simulink model "SpaceRobot"  (R2025b)
settings: Solver=ode4  StartTime=0.0  StopTime=8.5  FixedStep=0.01  RelTol=1e-5  AbsTol=1e-6
undefined symbols (not defined in the file or in its folder): d_safe, isdone_init, reward_init, Ts_agent, X, Y, Z
libraries: sm_lib x53, nesl_utility x34, rllib x1, sharedutil x1
(part 1 of 2)
settings Model: Creator=Deermste  LastModifiedBy=Deermste
settings ExplorerConfigSet: InternalSimMechanicsExplorerSettings="<ExplorerConfiguration><canonicalview>default</canonicalview><TilePanel><TileInfo><Tiles Columns=\"1\" Count=\"1\" Height=\"297\" Rows=\"1\" Width=\"493\"><Row Weight=\"1\"/><Column Weight=\"1\"/><Tile Height=\"1\" Width=\"1\" X=\"0\" Y=\"0\"/></Tiles></TileInfo><SceneInfo><SceneViewer><IsThisViewStd><IsStandardView>off</IsStandardView><StandardViewName>Front</StandardViewName></IsThisViewStd><BGColor><R>1</R><G>1</G><B>1</B><A>1</A></BGColor><Camera><DoPerspective>off</DoPerspective><Position><X>1.8433594980602974</X><Y>0.042277202971402056</Y><Z>13.278475546002786</Z></Position><Center><X>1.8433594980602974</X><Y>0.042277202971402056</Y><Z>0</Z></Center><Up><X>0</X><Y>1</Y><Z>0</Z></Up><XLim>1.9650781003092099</XLim><YLim>1.9650781003092099</YLim><ViewLimDist>0.01</ViewLimDist></Camera></SceneViewer></SceneInfo></TilePanel><MechEditorPanel><GfxPanelCameraMap/><Cameras/><VideoCreator><IncludeTiles>All</IncludeTiles><IncludeTime>on</IncludeTime><IncludeWorldFrame>off</IncludeWorldFrame><PlaybackSpeedRatio>1</PlaybackSpeedRatio><FrameRate>30</FrameRate><FrameSize>auto</FrameSize><VideoFormat>UncompressedAVI</VideoFormat></VideoCreator></MechEditorPanel><PlaybackSettings><PlaybackSpeedFactor>1</PlaybackSpeedFactor></PlaybackSettings></ExplorerConfiguration>"
settings ConfigComp: DVMaxProcessTime=300.0  DVMaxTestCaseSteps=10000.0  DVTestSuiteOptimization=Auto  DVAbsoluteTolerance=1.0e-5  DVDefectChecker=on  DVDetectOutOfBounds=on  DVMaxViolationSteps=20.0  DVModelReferenceHarness=on  DVHarnessSource=Signal Editor  DVActiveTab=0.0

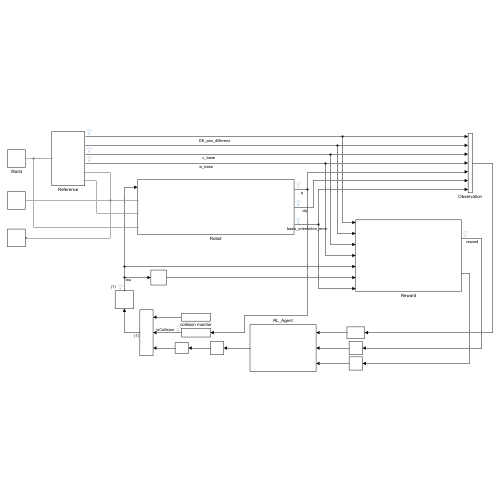
[thumbnail: Simulink's stored preview of the top-level diagram]
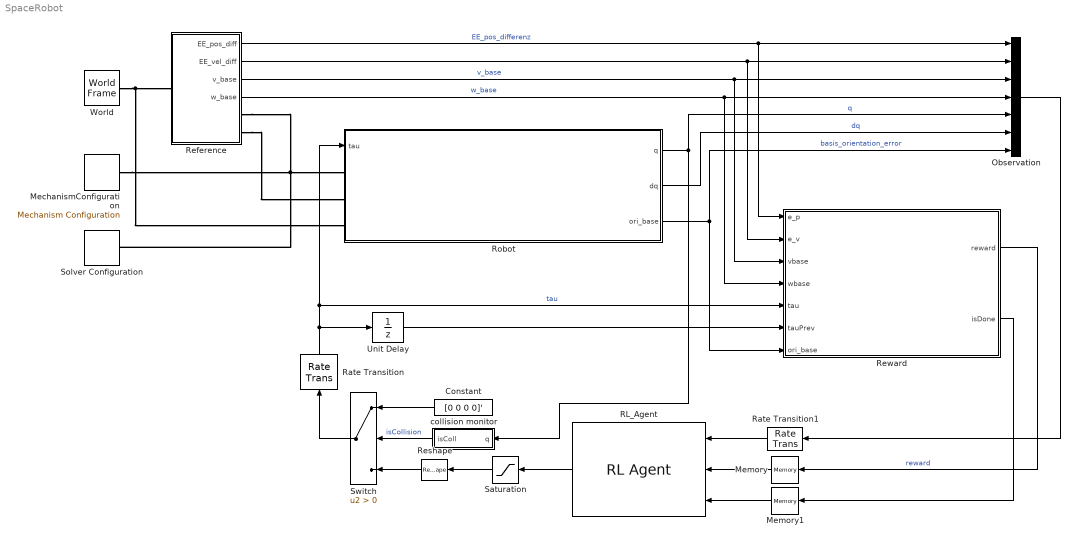
== system SpaceRobot ==
  Constant : Constant  Value=[0 0 0 0]'
  MechanismConfiguration : sm_lib/Utilities/Mechanism Configuration  UniformGravity=Constant  GravityVector=[0 0 0]  GravityVectorUnits=m/s^2  LinearizationDelta=0.001  JointModeTransitionNonlinearIterations=2
  Memory : Memory  InitialCondition=reward_init  InheritSampleTime=on
  Memory1 : Memory  InitialCondition=isdone_init  InheritSampleTime=on
  Observation : Mux  Inputs=7
  RL_Agent : rllib/RL Agent  Agent=agent  ExternalActionAsInput=off  ProvideLastAction=off  ProvideCumRwd=off  TreatAsDirectFeedthrough=on  UseStrictObservationDataTypes=off
  Rate Transition : RateTransition  OutPortSampleTime=Ts
  Rate Transition1 : RateTransition  OutPortSampleTime=Ts_agent
  Reference : Subsystem
  Reshape : Reshape  OutputDimensionality=Customize  OutputDimensions=[4, 1]
  Reward : Subsystem
  Robot : Subsystem
  Saturation : Saturate  UpperLimit=2  LowerLimit=-2
  Solver Configuration : nesl_utility/Solver Configuration  PhysicalDomain=network_engine_domain  SubClassName=solver  LeftPortType=input  RightPortType=generic  Tones=[]  Harmonics=[]  SimulateNoise=off  Profile=off  UseLocalSampling=off  EnableSwitchedLinearOptims=on  FrequencyDomain=off  UseCCode=off  RelTol=0.001  AbsTol=0.001  MinStep=1e-09  ToWorkspace=off  RevertToSquareIcSolve=off  NumHomotopyIterations=100  PhasorMode=off  PhasorModeNumHarmonics=1  ConsistencySolver=NEWTON_XTOL_AFTER_FTOL  IndexReductionMethod=DerivativeReplacement  DoDC=off  ResidualTolerance=1e-09  ConsistencyTolSource=GLOBAL  ConsistencyAbsTol=0.001  ConsistencyRelTol=0.001  ConsistencyTolFactor=0.001  UseLocalSolver=off  LocalSolverChoice=NE_BACKWARD_EULER_ADVANCER  ResolveIndetEquations=on  FunctionEvalNumThread=1  LocalSolverSampleTime=0.001  DoFixedCost=off  MaxNonlinIter=3  MaxModeIter=2  ComputeImpulses=off  ImpulseIterations=2  LinearAlgebra=auto  LinearAlgebraNumThread=0  EquationFormulation=NE_TIME_EF  DelaysMemoryBudget=1024  AutomaticFiltering=on  FilteringTimeConstant=0.001  PartitionStorageMethod=AS_NEEDED  PartitionMemoryBudget=1024  PartitionMethod=ROBUST  MultibodyUseLocalSolver=off  MultibodyLocalSolverChoice=ODE1  MultibodyLocalSolverSampleTime=0.001
  Switch : Switch  Criteria=u2 > Threshold  SaturateOnIntegerOverflow=off  InputSameDT=off
  Unit Delay : UnitDelay  InitialCondition=zeros(4,1)  SampleTime=-1  HasFrameUpgradeWarning=on
  World : sm_lib/Frames and Transforms/World Frame
  collision monitor : Subsystem
  wires:
  Unit Delay/1 -> Reward/6(tauPrev)
  Observation/1 -> Rate Transition1/1
  Reward/1(reward) -> Memory/1  "reward"
  Reward/2(isDone) -> Memory1/1
  Memory/1 -> RL_Agent/2
  Memory1/1 -> RL_Agent/3
  Robot/2(dq) -> Observation/6  "dq"
  Reference/2(EE_vel_diff) -> Reward/2(e_v), Observation/2
  Reference/1(EE_pos_diff) -> Reward/1(e_p), Observation/1  "EE_pos_differenz"
  Reference/4(w_base) -> Reward/4(wbase), Observation/4  "w_base"
  Reference/3(v_base) -> Reward/3(vbase), Observation/3  "v_base"
  Robot/3(ori_base) -> Reward/7(ori_base), Observation/7  "basis_orientation_error"
  Saturation/1 -> Reshape/1
  Rate Transition/1 -> Reward/5(tau), Robot/1(tau), Unit Delay/1  "tau"
  Rate Transition1/1 -> RL_Agent/1
  RL_Agent/1 -> Saturation/1
  Robot/1(q) -> collision monitor/1(q), Observation/5  "q"
  collision monitor/1(isColl) -> Switch/2  "isCollision"
  Switch/1 -> Rate Transition/1
  Constant/1 -> Switch/1
  Reshape/1 -> Switch/3
  connections:
  MechanismConfiguration/RConn1 -- Robot/LConn1 -- Solver Configuration/RConn1 -- Reference/RConn1
  World/RConn1 -- Robot/LConn3 -- Reference/LConn1
  Reference/RConn2 -- Robot/LConn2

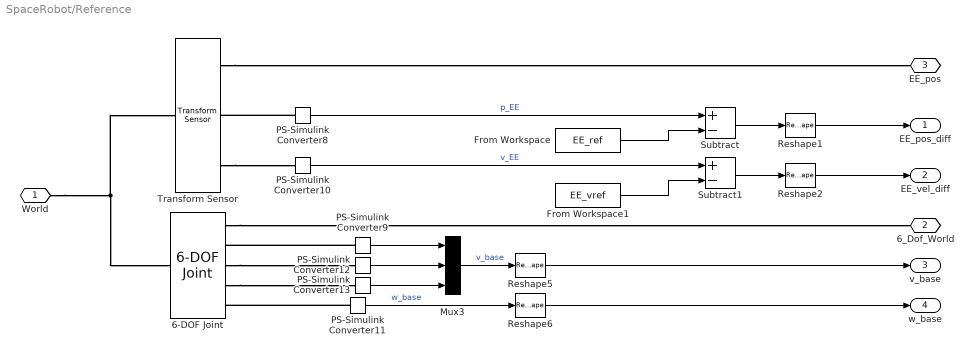
== system SpaceRobot/Reference ==
  6-DOF Joint : sm_lib/Joints/6-DOF Joint  JointMode=Normal  CompositeWrenchDir=FollowerOnBase  CompositeWrenchFrame=BaseFrame  SenseConstraintForce=off  SenseConstraintTorque=off  SenseTotalForce=off  SenseTotalTorque=off  PxPositionTargetSpecify=off  PxPositionTargetPriority=High  PxPositionTargetValue=0  PxPositionTargetValueUnits=m  PxVelocityTargetSpecify=off  PxVelocityTargetPriority=High  PxVelocityTargetValue=0  PxVelocityTargetValueUnits=m/s  PxEquilibriumPosition=0  PxEquilibriumPositionUnits=m  PxSpringStiffness=0  PxSpringStiffnessUnits=N/m  PxDampingCoefficient=0  PxDampingCoefficientUnits=N/(m/s)  PxLowerLimitSpecify=off  PxLowerLimitBound=-1  PxLowerLimitBoundUnits=m  PxLowerLimitStiffness=1e6  PxLowerLimitStiffnessUnits=N/m  PxLowerLimitDamping=1e3  PxLowerLimitDampingUnits=N/(m/s)  PxLowerLimitTransitionRegionWidth=1e-4  PxLowerLimitTransitionRegionWidthUnits=m  PxUpperLimitSpecify=off  PxUpperLimitBound=1  PxUpperLimitBoundUnits=m  PxUpperLimitStiffness=1e6  PxUpperLimitStiffnessUnits=N/m  PxUpperLimitDamping=1e3  PxUpperLimitDampingUnits=N/(m/s)  PxUpperLimitTransitionRegionWidth=1e-4  PxUpperLimitTransitionRegionWidthUnits=m  PxTorqueActuationMode=NoTorque  PxMotionActuationMode=ComputedMotion  PxSensePosition=off  PxSenseVelocity=on  PxSenseAcceleration=off  PxSenseTorqueForce=off  PxSenseLowerLimitTorqueForce=off  PxSenseUpperLimitTorqueForce=off  PyPositionTargetSpecify=off  PyPositionTargetPriority=High  PyPositionTargetValue=0  PyPositionTargetValueUnits=m  PyVelocityTargetSpecify=off  PyVelocityTargetPriority=High  PyVelocityTargetValue=0  PyVelocityTargetValueUnits=m/s  PyEquilibriumPosition=0  PyEquilibriumPositionUnits=m  PySpringStiffness=0  PySpringStiffnessUnits=N/m  PyDampingCoefficient=0  PyDampingCoefficientUnits=N/(m/s)  PyLowerLimitSpecify=off  PyLowerLimitBound=-1  PyLowerLimitBoundUnits=m  PyLowerLimitStiffness=1e6  PyLowerLimitStiffnessUnits=N/m  PyLowerLimitDamping=1e3  PyLowerLimitDampingUnits=N/(m/s)  PyLowerLimitTransitionRegionWidth=1e-4  PyLowerLimitTransitionRegionWidthUnits=m  PyUpperLimitSpecify=off  PyUpperLimitBound=1  PyUpperLimitBoundUnits=m  PyUpperLimitStiffness=1e6  PyUpperLimitStiffnessUnits=N/m  PyUpperLimitDamping=1e3  PyUpperLimitDampingUnits=N/(m/s)  PyUpperLimitTransitionRegionWidth=1e-4  PyUpperLimitTransitionRegionWidthUnits=m  PyTorqueActuationMode=NoTorque  PyMotionActuationMode=ComputedMotion  PySensePosition=off  PySenseVelocity=on  PySenseAcceleration=off  PySenseTorqueForce=off  PySenseLowerLimitTorqueForce=off  PySenseUpperLimitTorqueForce=off  PzPositionTargetSpecify=off  PzPositionTargetPriority=High  PzPositionTargetValue=0  PzPositionTargetValueUnits=m  PzVelocityTargetSpecify=off  PzVelocityTargetPriority=High  PzVelocityTargetValue=0  PzVelocityTargetValueUnits=m/s  PzEquilibriumPosition=0  PzEquilibriumPositionUnits=m  PzSpringStiffness=0  PzSpringStiffnessUnits=N/m  PzDampingCoefficient=0  PzDampingCoefficientUnits=N/(m/s)  PzLowerLimitSpecify=off  PzLowerLimitBound=-1  PzLowerLimitBoundUnits=m  PzLowerLimitStiffness=1e6  PzLowerLimitStiffnessUnits=N/m  PzLowerLimitDamping=1e3  PzLowerLimitDampingUnits=N/(m/s)  PzLowerLimitTransitionRegionWidth=1e-4  PzLowerLimitTransitionRegionWidthUnits=m  PzUpperLimitSpecify=off  PzUpperLimitBound=1  PzUpperLimitBoundUnits=m  PzUpperLimitStiffness=1e6  PzUpperLimitStiffnessUnits=N/m  PzUpperLimitDamping=1e3  PzUpperLimitDampingUnits=N/(m/s)  PzUpperLimitTransitionRegionWidth=1e-4  PzUpperLimitTransitionRegionWidthUnits=m  PzTorqueActuationMode=NoTorque  PzMotionActuationMode=ComputedMotion  PzSensePosition=off  PzSenseVelocity=on  PzSenseAcceleration=off  PzSenseTorqueForce=off  PzSenseLowerLimitTorqueForce=off  PzSenseUpperLimitTorqueForce=off  SphPositionTargetSpecify=off  SphPositionTargetPriority=High  SphPositionTargetRotationMethod=None  SphPositionTargetFollAlignAxisA=+X  SphPositionTargetBaseAlignAxisA=+Y  SphPositionTargetFollAlignAxisB=+Y  SphPositionTargetBaseAlignAxisB=+Z  SphPositionTargetRotationStandardAxis=+Z  SphPositionTargetRotationAngle=0  SphPositionTargetRotationAngleUnits=deg  SphPositionTargetRotationArbitraryAxis=[0 0 1]  SphPositionTargetRotationSequenceAxes=FollowerAxes  SphPositionTargetRotationSequence=XYX  SphPositionTargetRotationSequenceAngles=[0 0 0]  SphPositionTargetRotationSequenceAnglesUnits=deg  SphPositionTargetRotationMatrix=[1 0 0;0 1 0;0 0 1]  SphPositionTargetQuaternion=[1 0 0 0]  SphVelocityTargetSpecify=off  SphVelocityTargetPriority=High  SphVelocityTargetValue=[0 0 0]  SphVelocityTargetValueUnits=deg/s  SphVelocityTargetInFollowerFrame=on  SphEqPosRotationMethod=None  SphEqPosFollAlignAxisA=+X  SphEqPosBaseAlignAxisA=+Y  SphEqPosFollAlignAxisB=+Y  SphEqPosBaseAlignAxisB=+Z  SphEqPosRotationStandardAxis=+Z  SphEqPosRotationAngle=0  SphEqPosRotationAngleUnits=deg  SphEqPosRotationArbitraryAxis=[0 0 1]  SphEqPosRotationSequenceAxes=FollowerAxes  SphEqPosRotationSequence=XYX  SphEqPosRotationSequenceAngles=[0 0 0]  SphEqPosRotationSequenceAnglesUnits=deg  SphEqPosRotationMatrix=[1 0 0;0 1 0;0 0 1]  SphEqPosQuaternion=[1 0 0 0]  SphSpringStiffness=0  SphSpringStiffnessUnits=N*m/deg  SphDampingCoefficient=0  SphDampingCoefficientUnits=N*m/(deg/s)  SphLowerLimitSpecify=off  SphLowerLimitBound=15  SphLowerLimitBoundUnits=deg  SphLowerLimitStiffness=1e4  SphLowerLimitStiffnessUnits=N*m/deg  SphLowerLimitDamping=10  SphLowerLimitDampingUnits=N*m/(deg/s)  SphLowerLimitTransitionRegionWidth=0.1  SphLowerLimitTransitionRegionWidthUnits=deg  SphUpperLimitSpecify=off  SphUpperLimitBound=45  SphUpperLimitBoundUnits=deg  SphUpperLimitStiffness=1e4  SphUpperLimitStiffnessUnits=N*m/deg  SphUpperLimitDamping=10  SphUpperLimitDampingUnits=N*m/(deg/s)  SphUpperLimitTransitionRegionWidth=0.1  SphUpperLimitTransitionRegionWidthUnits=deg  SphTorqueActuationMode=NoTorque  SphActuateTorqueX=off  SphActuateTorqueY=off  SphActuateTorqueZ=off  SphActuateTorque=off  SphActuationFrame=BaseFrame  SphSensePosition=off  SphSenseVelocityX=off  SphSenseVelocityY=off  SphSenseVelocityZ=off  SphSenseVelocity=on  SphSenseAccelerationX=off  SphSenseAccelerationY=off  SphSenseAccelerationZ=off  SphSenseAcceleration=off  SphSenseLowerLimitTorqueMag=off  SphSenseUpperLimitTorqueMag=off  SphSensingFrame=BaseFrame
  From Workspace : FromWorkspace  VariableName=EE_ref
  From Workspace1 : FromWorkspace  VariableName=EE_vref
  Mux3 : Mux  Inputs=3
  PS-Simulink Converter{8..13} (6 alike) : nesl_utility/PS-Simulink Converter  PhysicalDomain=network_engine_domain  SubClassName=ps_output  LeftPortType=input  RightPortType=output  PseudoPeriodic=off  Frequencies=[]  VectorFormat=inherit  Unit=inherit  AffineConversion=off
  Reshape{1..2,5..6} (4 alike) : Reshape  OutputDimensionality=Customize  OutputDimensions=[3, 1]
  Subtract : Sum  Inputs=+-
  Subtract1 : Sum  Inputs=+-
  Transform Sensor : sm_lib/Frames and Transforms/Transform Sensor  MeasurementFrame=World  RotationSequence=XYX  SenseAngle=off  SenseAxis=off  SenseQ=off  SenseR=off  SenseRotationSequence=off  SenseOmegaX=off  SenseOmegaY=off  SenseOmegaZ=off  SenseOmega=off  SenseQDot=off  SenseRDot=off  SenseRotationSequenceDot=off  SenseAlphaX=off  SenseAlphaY=off  SenseAlphaZ=off  SenseAlpha=off  SenseQDDot=off  SenseRDDot=off  SenseX=off  SenseY=off  SenseZ=off  SenseXYZ=on  SenseRad=off  SenseAzim=off  SenseDist=off  SenseInc=off  SenseXDot=off  SenseYDot=off  SenseZDot=off  SenseXYZDot=on  SenseRadDot=off  SenseAzimDot=off  SenseDistDot=off  SenseIncDot=off  SenseXDDot=off  SenseYDDot=off  SenseZDDot=off  SenseXYZDDot=off  SenseRadDDot=off  SenseAzimDDot=off  SenseDistDDot=off  SenseIncDDot=off
  World : PMIOPort  Side=Left
  6_Dof_World : PMIOPort  Port=2  Side=Right
  EE_pos : PMIOPort  Port=3  Side=Right
  EE_pos_diff : Outport
  EE_vel_diff : Outport  Port=2
  v_base : Outport  Port=3
  w_base : Outport  Port=4
  wires:
  PS-Simulink Converter8/1 -> Subtract/1  "p_EE"
  PS-Simulink Converter11/1 -> Reshape6/1  "w_base"
  From Workspace1/1 -> Subtract1/2
  Mux3/1 -> Reshape5/1  "v_base"
  PS-Simulink Converter10/1 -> Subtract1/1  "v_EE"
  Reshape1/1 -> EE_pos_diff/1
  PS-Simulink Converter13/1 -> Mux3/3
  From Workspace/1 -> Subtract/2
  PS-Simulink Converter9/1 -> Mux3/1
  Subtract/1 -> Reshape1/1
  Subtract1/1 -> Reshape2/1
  PS-Simulink Converter12/1 -> Mux3/2
  Reshape5/1 -> v_base/1
  Reshape2/1 -> EE_vel_diff/1
  Reshape6/1 -> w_base/1
  connections:
  Transform Sensor/RConn3 -- PS-Simulink Converter10/LConn1
  6-DOF Joint/RConn3 -- PS-Simulink Converter12/LConn1
  World/RConn1 -- Transform Sensor/LConn1 -- 6-DOF Joint/LConn1
  PS-Simulink Converter11/LConn1 -- 6-DOF Joint/RConn5
  6-DOF Joint/RConn4 -- PS-Simulink Converter13/LConn1
  PS-Simulink Converter9/LConn1 -- 6-DOF Joint/RConn2
  PS-Simulink Converter8/LConn1 -- Transform Sensor/RConn2
  Transform Sensor/RConn1 -- EE_pos/RConn1
  6-DOF Joint/RConn1 -- 6_Dof_World/RConn1

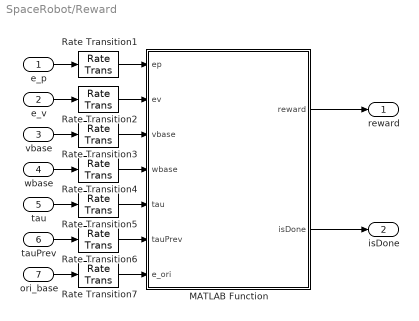
== system SpaceRobot/Reward ==
  e_p : Inport
  e_v : Inport  Port=2
  vbase : Inport  Port=3
  wbase : Inport  Port=4
  tau : Inport  Port=5
  tauPrev : Inport  Port=6
  ori_base : Inport  Port=7
  MATLAB Function : MATLAB Function  TreatAsAtomicUnit=on  SystemSampleTime=Ts_agent
  Rate Transition{1..7} (7 alike) : RateTransition  OutPortSampleTime=Ts_agent
  reward : Outport
  isDone : Outport  Port=2
  wires:
  MATLAB Function/1(reward) -> reward/1
  MATLAB Function/2(isDone) -> isDone/1
  e_p/1 -> Rate Transition1/1
  e_v/1 -> Rate Transition2/1
  vbase/1 -> Rate Transition3/1
  wbase/1 -> Rate Transition4/1
  tau/1 -> Rate Transition5/1
  tauPrev/1 -> Rate Transition6/1
  ori_base/1 -> Rate Transition7/1
  Rate Transition1/1 -> MATLAB Function/1(ep)
  Rate Transition2/1 -> MATLAB Function/2(ev)
  Rate Transition3/1 -> MATLAB Function/3(vbase)
  Rate Transition4/1 -> MATLAB Function/4(wbase)
  Rate Transition5/1 -> MATLAB Function/5(tau)
  Rate Transition6/1 -> MATLAB Function/6(tauPrev)
  Rate Transition7/1 -> MATLAB Function/7(e_ori)

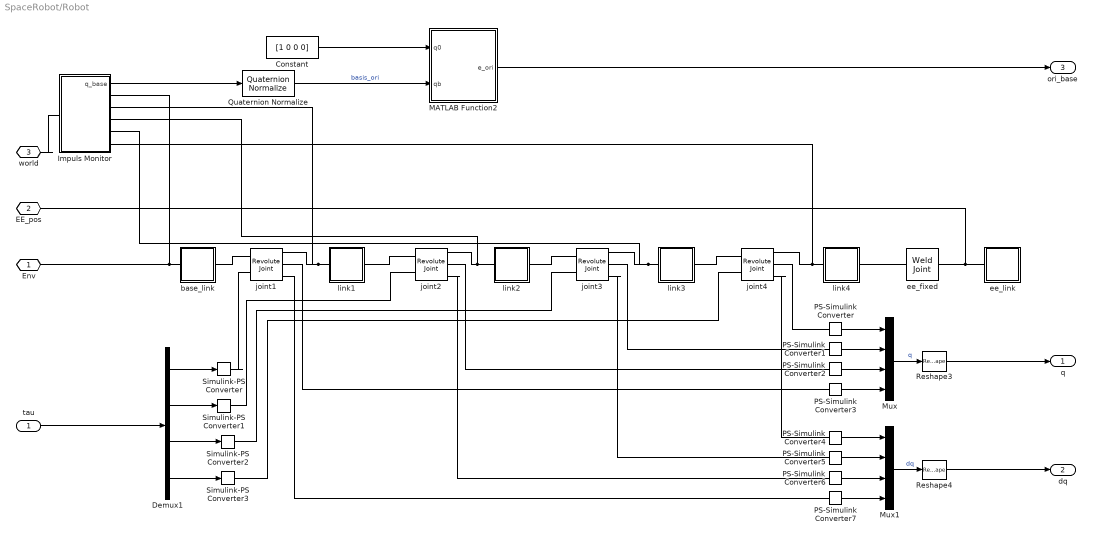
== system SpaceRobot/Robot ==
  tau : Inport
  Constant : Constant  Value=[1 0 0 0]
  Demux1 : Demux
  Impuls Monitor : Subsystem
  MATLAB Function2 : MATLAB Function  TreatAsAtomicUnit=on
  Mux : Mux
  Mux1 : Mux
  PS-Simulink Converter{,1..7} (8 alike) : nesl_utility/PS-Simulink Converter  PhysicalDomain=network_engine_domain  SubClassName=ps_output  LeftPortType=input  RightPortType=output  PseudoPeriodic=off  Frequencies=[]  VectorFormat=inherit  Unit=inherit  AffineConversion=off
  Quaternion Normalize : sharedutil/Quaternion Normalize  aMode=aMode
  Reshape3 : Reshape  OutputDimensionality=Customize  OutputDimensions=[4, 1]
  Reshape4 : Reshape  OutputDimensionality=Customize  OutputDimensions=[4, 1]
  Simulink-PS Converter{,1..3} (4 alike) : nesl_utility/Simulink-PS Converter  PhysicalDomain=network_engine_domain  SubClassName=ps_input  LeftPortType=input  RightPortType=output  PseudoPeriodic=off  Frequencies=[]  NoiseDistribution=none  NoiseParameters=[]  Unit=1  AffineConversion=off  FilteringAndDerivatives=provide  SimscapeFilterOrder=1  InputFilterTimeConstant=0.001  UdotUserProvided=0
  base_link : Subsystem
  ee_fixed : sm_lib/Joints/Weld Joint  JointMode=Normal  CompositeWrenchDir=FollowerOnBase  CompositeWrenchFrame=BaseFrame  SenseConstraintForce=off  SenseConstraintTorque=off  SenseTotalForce=off  SenseTotalTorque=off
  ee_link : Subsystem
  joint1 : sm_lib/Joints/Revolute Joint  JointMode=Normal  CompositeWrenchDir=FollowerOnBase  CompositeWrenchFrame=BaseFrame  SenseConstraintForce=off  SenseConstraintTorque=off  SenseTotalForce=off  SenseTotalTorque=off  PositionTargetSpecify=on  PositionTargetPriority=High  PositionTargetValue=0  PositionTargetValueUnits=deg  VelocityTargetSpecify=on  VelocityTargetPriority=High  VelocityTargetValue=0  VelocityTargetValueUnits=deg/s  EquilibriumPosition=0  EquilibriumPositionUnits=deg  SpringStiffness=0  SpringStiffnessUnits=N*m/deg  DampingCoefficient=1.5  DampingCoefficientUnits=N*m*s/rad  LowerLimitSpecify=on  LowerLimitBound=-85  LowerLimitBoundUnits=deg  LowerLimitStiffness=3000  LowerLimitStiffnessUnits=N*m/rad  LowerLimitDamping=40  LowerLimitDampingUnits=N*m*s/rad  LowerLimitTransitionRegionWidth=0.03  LowerLimitTransitionRegionWidthUnits=rad  UpperLimitSpecify=on  UpperLimitBound=85  UpperLimitBoundUnits=deg  UpperLimitStiffness=3000  UpperLimitStiffnessUnits=N*m/rad  UpperLimitDamping=40  UpperLimitDampingUnits=N*m*s/rad  UpperLimitTransitionRegionWidth=0.03  UpperLimitTransitionRegionWidthUnits=rad  TorqueActuationMode=InputTorque  MotionActuationMode=ComputedMotion  SensePosition=on  SenseVelocity=on  SenseAcceleration=off  SenseTorqueForce=off  SenseLowerLimitTorqueForce=off  SenseUpperLimitTorqueForce=off
  joint2 : sm_lib/Joints/Revolute Joint  JointMode=Normal  CompositeWrenchDir=FollowerOnBase  CompositeWrenchFrame=BaseFrame  SenseConstraintForce=off  SenseConstraintTorque=off  SenseTotalForce=off  SenseTotalTorque=off  PositionTargetSpecify=on  PositionTargetPriority=High  PositionTargetValue=0  PositionTargetValueUnits=deg  VelocityTargetSpecify=on  VelocityTargetPriority=High  VelocityTargetValue=0  VelocityTargetValueUnits=deg/s  EquilibriumPosition=0  EquilibriumPositionUnits=deg  SpringStiffness=0  SpringStiffnessUnits=N*m/deg  DampingCoefficient=1.5  DampingCoefficientUnits=N*m*s/rad  LowerLimitSpecify=on  LowerLimitBound=-170  LowerLimitBoundUnits=deg  LowerLimitStiffness=3000  LowerLimitStiffnessUnits=N*m/rad  LowerLimitDamping=40  LowerLimitDampingUnits=N*m*s/rad  LowerLimitTransitionRegionWidth=0.03  LowerLimitTransitionRegionWidthUnits=rad  UpperLimitSpecify=on  UpperLimitBound=170  UpperLimitBoundUnits=deg  UpperLimitStiffness=3000  UpperLimitStiffnessUnits=N*m/rad  UpperLimitDamping=40  UpperLimitDampingUnits=N*m*s/rad  UpperLimitTransitionRegionWidth=0.03  UpperLimitTransitionRegionWidthUnits=rad  TorqueActuationMode=InputTorque  MotionActuationMode=ComputedMotion  SensePosition=on  SenseVelocity=on  SenseAcceleration=off  SenseTorqueForce=off  SenseLowerLimitTorqueForce=off  SenseUpperLimitTorqueForce=off
  joint3 : sm_lib/Joints/Revolute Joint  JointMode=Normal  CompositeWrenchDir=FollowerOnBase  CompositeWrenchFrame=BaseFrame  SenseConstraintForce=off  SenseConstraintTorque=off  SenseTotalForce=off  SenseTotalTorque=off  PositionTargetSpecify=on  PositionTargetPriority=High  PositionTargetValue=0  PositionTargetValueUnits=deg  VelocityTargetSpecify=on  VelocityTargetPriority=High  VelocityTargetValue=0  VelocityTargetValueUnits=deg/s  EquilibriumPosition=0  EquilibriumPositionUnits=deg  SpringStiffness=0  SpringStiffnessUnits=N*m/deg  DampingCoefficient=1.5  DampingCoefficientUnits=N*m*s/rad  LowerLimitSpecify=on  LowerLimitBound=-170  LowerLimitBoundUnits=deg  LowerLimitStiffness=3000  LowerLimitStiffnessUnits=N*m/rad  LowerLimitDamping=40  LowerLimitDampingUnits=N*m*s/rad  LowerLimitTransitionRegionWidth=0.03  LowerLimitTransitionRegionWidthUnits=rad  UpperLimitSpecify=on  UpperLimitBound=170  UpperLimitBoundUnits=deg  UpperLimitStiffness=3000  UpperLimitStiffnessUnits=N*m/rad  UpperLimitDamping=40  UpperLimitDampingUnits=N*m*s/rad  UpperLimitTransitionRegionWidth=0.03  UpperLimitTransitionRegionWidthUnits=rad  TorqueActuationMode=InputTorque  MotionActuationMode=ComputedMotion  SensePosition=on  SenseVelocity=on  SenseAcceleration=off  SenseTorqueForce=off  SenseLowerLimitTorqueForce=off  SenseUpperLimitTorqueForce=off
  joint4 : sm_lib/Joints/Revolute Joint  JointMode=Normal  CompositeWrenchDir=FollowerOnBase  CompositeWrenchFrame=BaseFrame  SenseConstraintForce=off  SenseConstraintTorque=off  SenseTotalForce=off  SenseTotalTorque=off  PositionTargetSpecify=on  PositionTargetPriority=High  PositionTargetValue=0  PositionTargetValueUnits=deg  VelocityTargetSpecify=on  VelocityTargetPriority=High  VelocityTargetValue=0  VelocityTargetValueUnits=deg/s  EquilibriumPosition=0  EquilibriumPositionUnits=deg  SpringStiffness=0  SpringStiffnessUnits=N*m/deg  DampingCoefficient=1.5  DampingCoefficientUnits=N*m*s/rad  LowerLimitSpecify=on  LowerLimitBound=-170  LowerLimitBoundUnits=deg  LowerLimitStiffness=3000  LowerLimitStiffnessUnits=N*m/rad  LowerLimitDamping=40  LowerLimitDampingUnits=N*m*s/rad  LowerLimitTransitionRegionWidth=0.03  LowerLimitTransitionRegionWidthUnits=rad  UpperLimitSpecify=on  UpperLimitBound=170  UpperLimitBoundUnits=deg  UpperLimitStiffness=3000  UpperLimitStiffnessUnits=N*m/rad  UpperLimitDamping=40  UpperLimitDampingUnits=N*m*s/rad  UpperLimitTransitionRegionWidth=0.03  UpperLimitTransitionRegionWidthUnits=rad  TorqueActuationMode=InputTorque  MotionActuationMode=ComputedMotion  SensePosition=on  SenseVelocity=on  SenseAcceleration=off  SenseTorqueForce=off  SenseLowerLimitTorqueForce=off  SenseUpperLimitTorqueForce=off
  link1 : Subsystem
  link2 : Subsystem
  link3 : Subsystem
  link4 : Subsystem
  Env : PMIOPort  Side=Left
  EE_pos : PMIOPort  Port=2  Side=Left
  world : PMIOPort  Port=3  Side=Left
  q : Outport
  dq : Outport  Port=2
  ori_base : Outport  Port=3
  wires:
  Mux1/1 -> Reshape4/1  "dq"
  PS-Simulink Converter5/1 -> Mux1/2
  PS-Simulink Converter1/1 -> Mux/2
  PS-Simulink Converter2/1 -> Mux/3
  Demux1/1 -> Simulink-PS Converter/1
  Mux/1 -> Reshape3/1  "q"
  Reshape3/1 -> q/1
  PS-Simulink Converter/1 -> Mux/1
  PS-Simulink Converter4/1 -> Mux1/1
  Demux1/3 -> Simulink-PS Converter2/1
  Reshape4/1 -> dq/1
  Demux1/2 -> Simulink-PS Converter1/1
  Demux1/4 -> Simulink-PS Converter3/1
  PS-Simulink Converter3/1 -> Mux/4
  PS-Simulink Converter6/1 -> Mux1/3
  PS-Simulink Converter7/1 -> Mux1/4
  tau/1 -> Demux1/1
  Quaternion Normalize/1 -> MATLAB Function2/2(qb)  "basis_ori"
  Constant/1 -> MATLAB Function2/1(q0)
  MATLAB Function2/1(e_ori) -> ori_base/1
  Impuls Monitor/1(q_base) -> Quaternion Normalize/1
  connections:
  joint4/RConn2 -- PS-Simulink Converter/LConn1
  joint3/RConn2 -- PS-Simulink Converter1/LConn1
  Simulink-PS Converter1/RConn1 -- joint2/LConn2
  ee_fixed/LConn1 -- link4/RConn1
  joint3/LConn1 -- link2/RConn1
  joint4/RConn3 -- PS-Simulink Converter4/LConn1
  joint1/RConn2 -- PS-Simulink Converter3/LConn1
  joint3/RConn3 -- PS-Simulink Converter5/LConn1
  joint2/RConn1 -- Impuls Monitor/RConn3 -- link2/LConn1
  joint2/RConn2 -- PS-Simulink Converter2/LConn1
  joint1/RConn3 -- PS-Simulink Converter7/LConn1
  joint4/LConn1 -- link3/RConn1
  Simulink-PS Converter/RConn1 -- joint1/LConn2
  base_link/RConn1 -- joint1/LConn1
  Simulink-PS Converter3/RConn1 -- joint4/LConn2
  joint2/LConn1 -- link1/RConn1
  ee_link/LConn1 -- EE_pos/RConn1 -- ee_fixed/RConn1
  joint2/RConn3 -- PS-Simulink Converter6/LConn1
  Simulink-PS Converter2/RConn1 -- joint3/LConn2
  joint4/RConn1 -- Impuls Monitor/RConn5 -- link4/LConn1
  base_link/LConn1 -- Impuls Monitor/RConn1 -- Env/RConn1
  link3/LConn1 -- Impuls Monitor/RConn4 -- joint3/RConn1
  link1/LConn1 -- Impuls Monitor/RConn2 -- joint1/RConn1
  world/RConn1 -- Impuls Monitor/LConn1

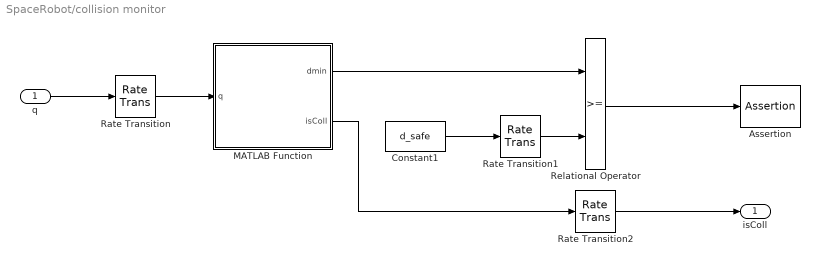
== system SpaceRobot/collision monitor ==
  q : Inport
  Assertion : Assertion  AssertionFailFcn="\"Collision detected\""  StopWhenAssertionFail=off
  Constant1 : Constant  Value=d_safe
  MATLAB Function : MATLAB Function  TreatAsAtomicUnit=on
  Rate Transition : RateTransition  OutPortSampleTime=Ts_agent
  Rate Transition1 : RateTransition  OutPortSampleTime=Ts_agent
  Rate Transition2 : RateTransition  OutPortSampleTime=Ts_agent
  Relational Operator : RelationalOperator  OutDataTypeStr=boolean  RndMeth=Simplest  InputSameDT=off
  isColl : Outport
  wires:
  Constant1/1 -> Rate Transition1/1
  q/1 -> Rate Transition/1
  MATLAB Function/1(dmin) -> Relational Operator/1
  Rate Transition/1 -> MATLAB Function/1(q)
  Rate Transition1/1 -> Relational Operator/2
  MATLAB Function/2(isColl) -> Rate Transition2/1
  Relational Operator/1 -> Assertion/1
  Rate Transition2/1 -> isColl/1

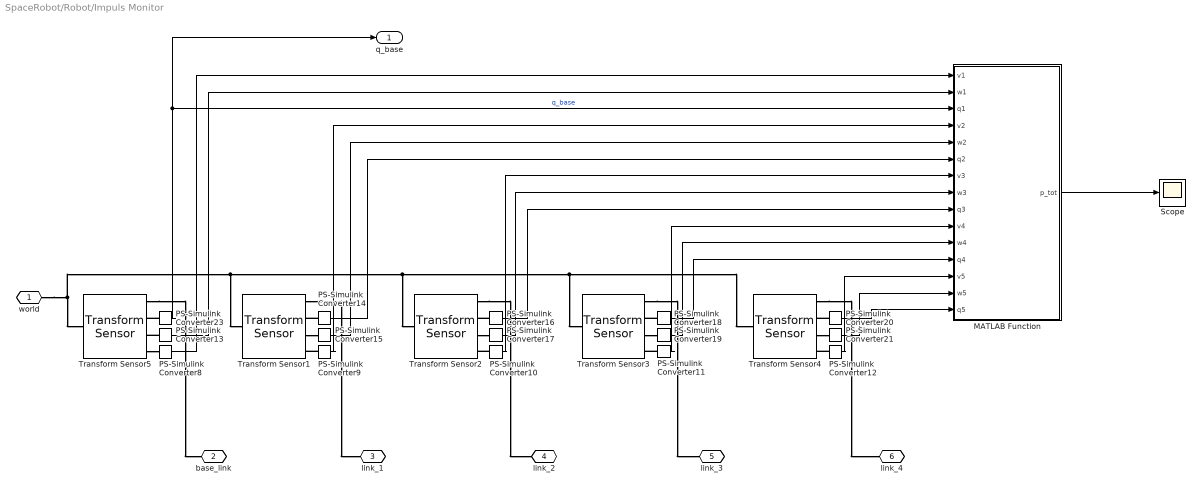
== system SpaceRobot/Robot/Impuls Monitor ==
  MATLAB Function : MATLAB Function  TreatAsAtomicUnit=on
  PS-Simulink Converter{8..21,23} (15 alike) : nesl_utility/PS-Simulink Converter  PhysicalDomain=network_engine_domain  SubClassName=ps_output  LeftPortType=input  RightPortType=output  PseudoPeriodic=off  Frequencies=[]  VectorFormat=inherit  Unit=inherit  AffineConversion=off
  Scope : Scope
      settings: ActiveDisplayYMinimum=-4.1636038465302455E-5  ActiveDisplayYMaximum=3.5566565679044735E-5
  Transform Sensor{1..5} (5 alike) : sm_lib/Frames and Transforms/Transform Sensor  MeasurementFrame=World  RotationSequence=XYX  SenseAngle=off  SenseAxis=off  SenseQ=on  SenseR=off  SenseRotationSequence=off  SenseOmegaX=off  SenseOmegaY=off  SenseOmegaZ=off  SenseOmega=on  SenseQDot=off  SenseRDot=off  SenseRotationSequenceDot=off  SenseAlphaX=off  SenseAlphaY=off  SenseAlphaZ=off  SenseAlpha=off  SenseQDDot=off  SenseRDDot=off  SenseX=off  SenseY=off  SenseZ=off  SenseXYZ=off  SenseRad=off  SenseAzim=off  SenseDist=off  SenseInc=off  SenseXDot=off  SenseYDot=off  SenseZDot=off  SenseXYZDot=on  SenseRadDot=off  SenseAzimDot=off  SenseDistDot=off  SenseIncDot=off  SenseXDDot=off  SenseYDDot=off  SenseZDDot=off  SenseXYZDDot=off  SenseRadDDot=off  SenseAzimDDot=off  SenseDistDDot=off  SenseIncDDot=off
  world : PMIOPort  Side=Left
  base_link : PMIOPort  Port=2  Side=Right
  link_1 : PMIOPort  Port=3  Side=Right
  link_2 : PMIOPort  Port=4  Side=Right
  link_3 : PMIOPort  Port=5  Side=Right
  link_4 : PMIOPort  Port=6  Side=Right
  q_base : Outport
  wires:
  PS-Simulink Converter23/1 -> q_base/1, MATLAB Function/3(q1)  "q_base"
  PS-Simulink Converter9/1 -> MATLAB Function/4(v2)
  PS-Simulink Converter18/1 -> MATLAB Function/12(q4)
  PS-Simulink Converter8/1 -> MATLAB Function/1(v1)
  PS-Simulink Converter12/1 -> MATLAB Function/13(v5)
  PS-Simulink Converter20/1 -> MATLAB Function/15(q5)
  PS-Simulink Converter14/1 -> MATLAB Function/6(q2)
  PS-Simulink Converter10/1 -> MATLAB Function/7(v3)
  PS-Simulink Converter11/1 -> MATLAB Function/10(v4)
  PS-Simulink Converter21/1 -> MATLAB Function/14(w5)
  PS-Simulink Converter19/1 -> MATLAB Function/11(w4)
  PS-Simulink Converter16/1 -> MATLAB Function/9(q3)
  MATLAB Function/1(p_tot) -> Scope/1
  PS-Simulink Converter15/1 -> MATLAB Function/5(w2)
  PS-Simulink Converter17/1 -> MATLAB Function/8(w3)
  PS-Simulink Converter13/1 -> MATLAB Function/2(w1)
  connections:
  PS-Simulink Converter23/LConn1 -- Transform Sensor5/RConn2
  PS-Simulink Converter9/LConn1 -- Transform Sensor1/RConn4
  world/RConn1 -- Transform Sensor5/LConn1 -- Transform Sensor4/LConn1 -- Transform Sensor3/LConn1 -- Transform Sensor2/LConn1 -- Transform Sensor1/LConn1
  Transform Sensor5/RConn1 -- base_link/RConn1
  Transform Sensor4/RConn1 -- link_4/RConn1
  PS-Simulink Converter10/LConn1 -- Transform Sensor2/RConn4
  PS-Simulink Converter16/LConn1 -- Transform Sensor2/RConn2
  PS-Simulink Converter12/LConn1 -- Transform Sensor4/RConn4
  Transform Sensor5/RConn4 -- PS-Simulink Converter8/LConn1
  PS-Simulink Converter20/LConn1 -- Transform Sensor4/RConn2
  PS-Simulink Converter11/LConn1 -- Transform Sensor3/RConn4
  PS-Simulink Converter14/LConn1 -- Transform Sensor1/RConn2
  Transform Sensor1/RConn3 -- PS-Simulink Converter15/LConn1
  Transform Sensor1/RConn1 -- link_1/RConn1
  PS-Simulink Converter13/LConn1 -- Transform Sensor5/RConn3
  PS-Simulink Converter18/LConn1 -- Transform Sensor3/RConn2
  Transform Sensor2/RConn3 -- PS-Simulink Converter17/LConn1
  Transform Sensor4/RConn3 -- PS-Simulink Converter21/LConn1
  Transform Sensor3/RConn3 -- PS-Simulink Converter19/LConn1
  Transform Sensor2/RConn1 -- link_2/RConn1
  Transform Sensor3/RConn1 -- link_3/RConn1

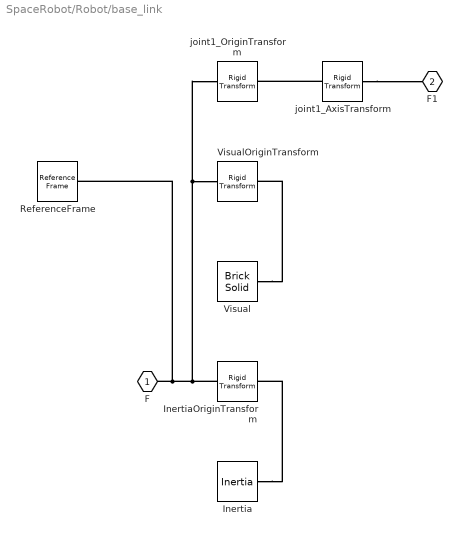
== system SpaceRobot/Robot/base_link ==
  Inertia : sm_lib/Body Elements/Inertia  InertiaType=Custom  Mass=5  MassUnits=kg  CenterOfMass=[0, 0, 0]  CenterOfMassUnits=m  MomentsOfInertia=[1 1, 1]  MomentsOfInertiaUnits=kg*m^2  ProductsOfInertia=[0, 0, 0]  ProductsOfInertiaUnits=kg*m^2  GraphicType=None  MarkerShape=Inertia  MarkerSize=20  GraphicVisPropType=SimpleVisualProperties  GraphicDiffuseColor=[0.5 0.5 0.5]  GraphicOpacity=1  GraphicSpecularColor=[0.5 0.5 0.5 1.0]  GraphicAmbientColor=[0.15 0.15 0.15 1.0]  GraphicEmissiveColor=[0.0 0.0 0.0 1.0]  GraphicShininess=75
  InertiaOriginTransform : sm_lib/Frames and Transforms/Rigid Transform  RotationMethod=RotationSequence  FollAlignAxisA=+X  BaseAlignAxisA=+Y  FollAlignAxisB=+Y  BaseAlignAxisB=+Z  RotationStandardAxis=+Z  RotationAngle=0  RotationAngleUnits=deg  RotationArbitraryAxis=[0 0 1]  RotationSequenceAxes=BaseAxes  RotationSequence=XYZ  RotationSequenceAngles=[0, 0, 0]  RotationSequenceAnglesUnits=rad  RotationMatrix=[1 0 0;0 1 0;0 0 1]  Quaternion=[1 0 0 0]  TranslationMethod=Cartesian  TranslationCartesianOffset=[0, 0, 0]  TranslationCartesianOffsetUnits=m  TranslationStandardAxis=+Z  TranslationStandardOffset=0  TranslationStandardOffsetUnits=m  TranslationROffset=0  TranslationROffsetUnits=m  TranslationThetaOffset=0  TranslationThetaOffsetUnits=deg  TranslationZOffset=0  TranslationZOffsetUnits=m
  ReferenceFrame : sm_lib/Frames and Transforms/Reference Frame
  Visual : sm_lib/Body Elements/Brick Solid  BrickDimensions=[1, 1, 1]  BrickDimensionsUnits=m  ExportEntireGeometry=off  InertiaType=Custom  BasedOnType=Density  Density=1000  DensityUnits=kg/m^3  Mass=5  MassUnits=kg  CenterOfMass=[0, 0, 0]  CenterOfMassUnits=m  MomentsOfInertia=[1, 1, 1]  MomentsOfInertiaUnits=kg*m^2  ProductsOfInertia=[0, 0, 0]  ProductsOfInertiaUnits=kg*m^2  GraphicType=FromGeometry  MarkerShape=Sphere  MarkerSize=10  GraphicVisPropType=SimpleVisualProperties  GraphicDiffuseColor=[0.2, 0.2, 0.8]  GraphicOpacity=1  GraphicSpecularColor=[0.5 0.5 0.5 1.0]  GraphicAmbientColor=[0.15 0.15 0.15 1.0]  GraphicEmissiveColor=[0.0 0.0 0.0 1.0]  GraphicShininess=75  DoExposeReferenceFrame=on  SerializedFrames=<Frames/>
  VisualOriginTransform : sm_lib/Frames and Transforms/Rigid Transform  RotationMethod=RotationSequence  FollAlignAxisA=+X  BaseAlignAxisA=+Y  FollAlignAxisB=+Y  BaseAlignAxisB=+Z  RotationStandardAxis=+Z  RotationAngle=0  RotationAngleUnits=deg  RotationArbitraryAxis=[0 0 1]  RotationSequenceAxes=BaseAxes  RotationSequence=XYZ  RotationSequenceAngles=[0, 0, 0]  RotationSequenceAnglesUnits=rad  RotationMatrix=[1 0 0;0 1 0;0 0 1]  Quaternion=[1 0 0 0]  TranslationMethod=Cartesian  TranslationCartesianOffset=[0, 0, 0]  TranslationCartesianOffsetUnits=m  TranslationStandardAxis=+Z  TranslationStandardOffset=0  TranslationStandardOffsetUnits=m  TranslationROffset=0  TranslationROffsetUnits=m  TranslationThetaOffset=0  TranslationThetaOffsetUnits=deg  TranslationZOffset=0  TranslationZOffsetUnits=m
  joint1_AxisTransform : sm_lib/Frames and Transforms/Rigid Transform  RotationMethod=ArbitraryAxis  FollAlignAxisA=+X  BaseAlignAxisA=+Y  FollAlignAxisB=+Y  BaseAlignAxisB=+Z  RotationStandardAxis=+Z  RotationAngle=0  RotationAngleUnits=rad  RotationArbitraryAxis=[1, 0, 0]  RotationSequenceAxes=FollowerAxes  RotationSequence=XYX  RotationSequenceAngles=[0 0 0]  RotationSequenceAnglesUnits=deg  RotationMatrix=[1 0 0;0 1 0;0 0 1]  Quaternion=[1 0 0 0]  TranslationMethod=Cartesian  TranslationCartesianOffset=[0, 0, 0]  TranslationCartesianOffsetUnits=m  TranslationStandardAxis=+Z  TranslationStandardOffset=0  TranslationStandardOffsetUnits=m  TranslationROffset=0  TranslationROffsetUnits=m  TranslationThetaOffset=0  TranslationThetaOffsetUnits=deg  TranslationZOffset=0  TranslationZOffsetUnits=m
  joint1_OriginTransform : sm_lib/Frames and Transforms/Rigid Transform  RotationMethod=RotationSequence  FollAlignAxisA=+X  BaseAlignAxisA=+Y  FollAlignAxisB=+Y  BaseAlignAxisB=+Z  RotationStandardAxis=+Z  RotationAngle=0  RotationAngleUnits=deg  RotationArbitraryAxis=[0 0 1]  RotationSequenceAxes=BaseAxes  RotationSequence=XYZ  RotationSequenceAngles=[0, 0, 0]  RotationSequenceAnglesUnits=rad  RotationMatrix=[1 0 0;0 1 0;0 0 1]  Quaternion=[1 0 0 0]  TranslationMethod=Cartesian  TranslationCartesianOffset=[0.5, 0, 0]  TranslationCartesianOffsetUnits=m  TranslationStandardAxis=+Z  TranslationStandardOffset=0  TranslationStandardOffsetUnits=m  TranslationROffset=0  TranslationROffsetUnits=m  TranslationThetaOffset=0  TranslationThetaOffsetUnits=deg  TranslationZOffset=0  TranslationZOffsetUnits=m
  F : PMIOPort  Side=Left
  F1 : PMIOPort  Port=2  Side=Right
  connections:
  Inertia/RConn1 -- InertiaOriginTransform/RConn1
  ReferenceFrame/RConn1 -- InertiaOriginTransform/LConn1 -- VisualOriginTransform/LConn1 -- joint1_OriginTransform/LConn1 -- F/RConn1
  Visual/RConn1 -- VisualOriginTransform/RConn1
  joint1_AxisTransform/RConn1 -- F1/RConn1
  joint1_AxisTransform/LConn1 -- joint1_OriginTransform/RConn1

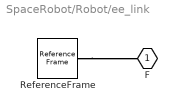
== system SpaceRobot/Robot/ee_link ==
  ReferenceFrame : sm_lib/Frames and Transforms/Reference Frame
  F : PMIOPort  Side=Left
  connections:
  ReferenceFrame/RConn1 -- F/RConn1

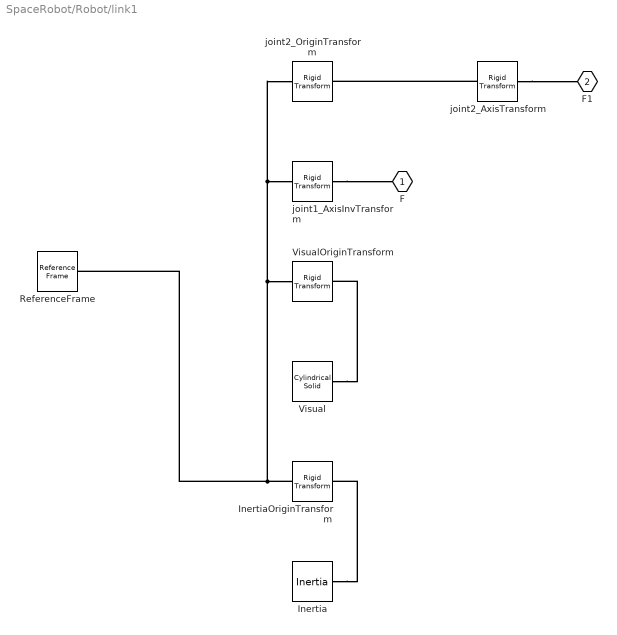
== system SpaceRobot/Robot/link1 ==
  Inertia : sm_lib/Body Elements/Inertia  InertiaType=Custom  Mass=1  MassUnits=kg  CenterOfMass=[0, 0, 0]  CenterOfMassUnits=m  MomentsOfInertia=[0.1, 0.1, 0.1]  MomentsOfInertiaUnits=kg*m^2  ProductsOfInertia=[0, 0, 0]  ProductsOfInertiaUnits=kg*m^2  GraphicType=None  MarkerShape=Inertia  MarkerSize=20  GraphicVisPropType=SimpleVisualProperties  GraphicDiffuseColor=[0.5 0.5 0.5]  GraphicOpacity=1  GraphicSpecularColor=[0.5 0.5 0.5 1.0]  GraphicAmbientColor=[0.15 0.15 0.15 1.0]  GraphicEmissiveColor=[0.0 0.0 0.0 1.0]  GraphicShininess=75
  InertiaOriginTransform : sm_lib/Frames and Transforms/Rigid Transform  RotationMethod=RotationSequence  FollAlignAxisA=+X  BaseAlignAxisA=+Y  FollAlignAxisB=+Y  BaseAlignAxisB=+Z  RotationStandardAxis=+Z  RotationAngle=0  RotationAngleUnits=deg  RotationArbitraryAxis=[0 0 1]  RotationSequenceAxes=BaseAxes  RotationSequence=XYZ  RotationSequenceAngles=[0, 0, 0]  RotationSequenceAnglesUnits=rad  RotationMatrix=[1 0 0;0 1 0;0 0 1]  Quaternion=[1 0 0 0]  TranslationMethod=Cartesian  TranslationCartesianOffset=[0.5, 0, 0]  TranslationCartesianOffsetUnits=m  TranslationStandardAxis=+Z  TranslationStandardOffset=0  TranslationStandardOffsetUnits=m  TranslationROffset=0  TranslationROffsetUnits=m  TranslationThetaOffset=0  TranslationThetaOffsetUnits=deg  TranslationZOffset=0  TranslationZOffsetUnits=m
  ReferenceFrame : sm_lib/Frames and Transforms/Reference Frame
  Visual : sm_lib/Body Elements/Cylindrical Solid  CylinderRadius=0.05  CylinderRadiusUnits=m  CylinderLength=1  CylinderLengthUnits=m  ExportEntireGeometry=off  InertiaType=Custom  BasedOnType=Density  Density=1000  DensityUnits=kg/m^3  Mass=1  MassUnits=kg  CenterOfMass=[0, 0, 0]  CenterOfMassUnits=m  MomentsOfInertia=[0.1, 0.1, 0.1]  MomentsOfInertiaUnits=kg*m^2  ProductsOfInertia=[0, 0, 0]  ProductsOfInertiaUnits=kg*m^2  GraphicType=FromGeometry  MarkerShape=Sphere  MarkerSize=10  GraphicVisPropType=SimpleVisualProperties  GraphicDiffuseColor=[0.5, 0.5, 0.5]  GraphicOpacity=1  GraphicSpecularColor=[0.5 0.5 0.5 1.0]  GraphicAmbientColor=[0.15 0.15 0.15 1.0]  GraphicEmissiveColor=[0.0 0.0 0.0 1.0]  GraphicShininess=75  DoExposeReferenceFrame=on  SerializedFrames=<Frames/>
  VisualOriginTransform : sm_lib/Frames and Transforms/Rigid Transform  RotationMethod=RotationSequence  FollAlignAxisA=+X  BaseAlignAxisA=+Y  FollAlignAxisB=+Y  BaseAlignAxisB=+Z  RotationStandardAxis=+Z  RotationAngle=0  RotationAngleUnits=deg  RotationArbitraryAxis=[0 0 1]  RotationSequenceAxes=BaseAxes  RotationSequence=XYZ  RotationSequenceAngles=[0, 1.5708, 0]  RotationSequenceAnglesUnits=rad  RotationMatrix=[1 0 0;0 1 0;0 0 1]  Quaternion=[1 0 0 0]  TranslationMethod=Cartesian  TranslationCartesianOffset=[0.5, 0, 0]  TranslationCartesianOffsetUnits=m  TranslationStandardAxis=+Z  TranslationStandardOffset=0  TranslationStandardOffsetUnits=m  TranslationROffset=0  TranslationROffsetUnits=m  TranslationThetaOffset=0  TranslationThetaOffsetUnits=deg  TranslationZOffset=0  TranslationZOffsetUnits=m
  joint1_AxisInvTransform : sm_lib/Frames and Transforms/Rigid Transform  RotationMethod=ArbitraryAxis  FollAlignAxisA=+X  BaseAlignAxisA=+Y  FollAlignAxisB=+Y  BaseAlignAxisB=+Z  RotationStandardAxis=+Z  RotationAngle=0  RotationAngleUnits=rad  RotationArbitraryAxis=[1, 0, 0]  RotationSequenceAxes=FollowerAxes  RotationSequence=XYX  RotationSequenceAngles=[0 0 0]  RotationSequenceAnglesUnits=deg  RotationMatrix=[1 0 0;0 1 0;0 0 1]  Quaternion=[1 0 0 0]  TranslationMethod=Cartesian  TranslationCartesianOffset=[0, 0, 0]  TranslationCartesianOffsetUnits=m  TranslationStandardAxis=+Z  TranslationStandardOffset=0  TranslationStandardOffsetUnits=m  TranslationROffset=0  TranslationROffsetUnits=m  TranslationThetaOffset=0  TranslationThetaOffsetUnits=deg  TranslationZOffset=0  TranslationZOffsetUnits=m
  joint2_AxisTransform : sm_lib/Frames and Transforms/Rigid Transform  RotationMethod=ArbitraryAxis  FollAlignAxisA=+X  BaseAlignAxisA=+Y  FollAlignAxisB=+Y  BaseAlignAxisB=+Z  RotationStandardAxis=+Z  RotationAngle=0  RotationAngleUnits=rad  RotationArbitraryAxis=[1, 0, 0]  RotationSequenceAxes=FollowerAxes  RotationSequence=XYX  RotationSequenceAngles=[0 0 0]  RotationSequenceAnglesUnits=deg  RotationMatrix=[1 0 0;0 1 0;0 0 1]  Quaternion=[1 0 0 0]  TranslationMethod=Cartesian  TranslationCartesianOffset=[0, 0, 0]  TranslationCartesianOffsetUnits=m  TranslationStandardAxis=+Z  TranslationStandardOffset=0  TranslationStandardOffsetUnits=m  TranslationROffset=0  TranslationROffsetUnits=m  TranslationThetaOffset=0  TranslationThetaOffsetUnits=deg  TranslationZOffset=0  TranslationZOffsetUnits=m
  joint2_OriginTransform : sm_lib/Frames and Transforms/Rigid Transform  RotationMethod=RotationSequence  FollAlignAxisA=+X  BaseAlignAxisA=+Y  FollAlignAxisB=+Y  BaseAlignAxisB=+Z  RotationStandardAxis=+Z  RotationAngle=0  RotationAngleUnits=deg  RotationArbitraryAxis=[0 0 1]  RotationSequenceAxes=BaseAxes  RotationSequence=XYZ  RotationSequenceAngles=[0, 0, 0]  RotationSequenceAnglesUnits=rad  RotationMatrix=[1 0 0;0 1 0;0 0 1]  Quaternion=[1 0 0 0]  TranslationMethod=Cartesian  TranslationCartesianOffset=[1, 0, 0]  TranslationCartesianOffsetUnits=m  TranslationStandardAxis=+Z  TranslationStandardOffset=0  TranslationStandardOffsetUnits=m  TranslationROffset=0  TranslationROffsetUnits=m  TranslationThetaOffset=0  TranslationThetaOffsetUnits=deg  TranslationZOffset=0  TranslationZOffsetUnits=m
  F : PMIOPort  Side=Left
  F1 : PMIOPort  Port=2  Side=Right
  connections:
  Inertia/RConn1 -- InertiaOriginTransform/RConn1
  ReferenceFrame/RConn1 -- InertiaOriginTransform/LConn1 -- joint1_AxisInvTransform/LConn1 -- joint2_OriginTransform/LConn1 -- VisualOriginTransform/LConn1
  Visual/RConn1 -- VisualOriginTransform/RConn1
  joint1_AxisInvTransform/RConn1 -- F/RConn1
  joint2_AxisTransform/RConn1 -- F1/RConn1
  joint2_AxisTransform/LConn1 -- joint2_OriginTransform/RConn1

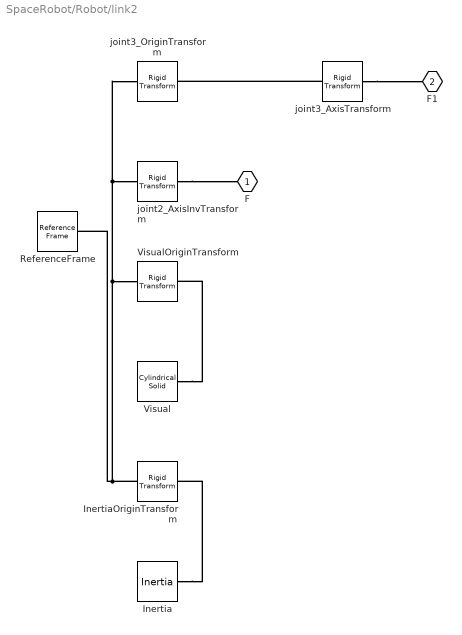
== system SpaceRobot/Robot/link2 ==
  Inertia : sm_lib/Body Elements/Inertia  InertiaType=Custom  Mass=1  MassUnits=kg  CenterOfMass=[0, 0, 0]  CenterOfMassUnits=m  MomentsOfInertia=[0.1, 0.1, 0.1]  MomentsOfInertiaUnits=kg*m^2  ProductsOfInertia=[0, 0, 0]  ProductsOfInertiaUnits=kg*m^2  GraphicType=None  MarkerShape=Inertia  MarkerSize=20  GraphicVisPropType=SimpleVisualProperties  GraphicDiffuseColor=[0.5 0.5 0.5]  GraphicOpacity=1  GraphicSpecularColor=[0.5 0.5 0.5 1.0]  GraphicAmbientColor=[0.15 0.15 0.15 1.0]  GraphicEmissiveColor=[0.0 0.0 0.0 1.0]  GraphicShininess=75
  InertiaOriginTransform : sm_lib/Frames and Transforms/Rigid Transform  RotationMethod=RotationSequence  FollAlignAxisA=+X  BaseAlignAxisA=+Y  FollAlignAxisB=+Y  BaseAlignAxisB=+Z  RotationStandardAxis=+Z  RotationAngle=0  RotationAngleUnits=deg  RotationArbitraryAxis=[0 0 1]  RotationSequenceAxes=BaseAxes  RotationSequence=XYZ  RotationSequenceAngles=[0, 0, 0]  RotationSequenceAnglesUnits=rad  RotationMatrix=[1 0 0;0 1 0;0 0 1]  Quaternion=[1 0 0 0]  TranslationMethod=Cartesian  TranslationCartesianOffset=[0.5, 0, 0]  TranslationCartesianOffsetUnits=m  TranslationStandardAxis=+Z  TranslationStandardOffset=0  TranslationStandardOffsetUnits=m  TranslationROffset=0  TranslationROffsetUnits=m  TranslationThetaOffset=0  TranslationThetaOffsetUnits=deg  TranslationZOffset=0  TranslationZOffsetUnits=m
  ReferenceFrame : sm_lib/Frames and Transforms/Reference Frame
  Visual : sm_lib/Body Elements/Cylindrical Solid  CylinderRadius=0.05  CylinderRadiusUnits=m  CylinderLength=1  CylinderLengthUnits=m  ExportEntireGeometry=off  InertiaType=Custom  BasedOnType=Density  Density=1000  DensityUnits=kg/m^3  Mass=1  MassUnits=kg  CenterOfMass=[0, 0, 0]  CenterOfMassUnits=m  MomentsOfInertia=[0.1, 0.1, 0.1]  MomentsOfInertiaUnits=kg*m^2  ProductsOfInertia=[0, 0, 0]  ProductsOfInertiaUnits=kg*m^2  GraphicType=FromGeometry  MarkerShape=Sphere  MarkerSize=10  GraphicVisPropType=SimpleVisualProperties  GraphicDiffuseColor=[0.6, 0.6, 0.6]  GraphicOpacity=1  GraphicSpecularColor=[0.5 0.5 0.5 1.0]  GraphicAmbientColor=[0.15 0.15 0.15 1.0]  GraphicEmissiveColor=[0.0 0.0 0.0 1.0]  GraphicShininess=75  DoExposeReferenceFrame=on  SerializedFrames=<Frames/>
  VisualOriginTransform : sm_lib/Frames and Transforms/Rigid Transform  RotationMethod=RotationSequence  FollAlignAxisA=+X  BaseAlignAxisA=+Y  FollAlignAxisB=+Y  BaseAlignAxisB=+Z  RotationStandardAxis=+Z  RotationAngle=0  RotationAngleUnits=deg  RotationArbitraryAxis=[0 0 1]  RotationSequenceAxes=BaseAxes  RotationSequence=XYZ  RotationSequenceAngles=[0, 1.5708, 0]  RotationSequenceAnglesUnits=rad  RotationMatrix=[1 0 0;0 1 0;0 0 1]  Quaternion=[1 0 0 0]  TranslationMethod=Cartesian  TranslationCartesianOffset=[0.5, 0, 0]  TranslationCartesianOffsetUnits=m  TranslationStandardAxis=+Z  TranslationStandardOffset=0  TranslationStandardOffsetUnits=m  TranslationROffset=0  TranslationROffsetUnits=m  TranslationThetaOffset=0  TranslationThetaOffsetUnits=deg  TranslationZOffset=0  TranslationZOffsetUnits=m
  joint2_AxisInvTransform : sm_lib/Frames and Transforms/Rigid Transform  RotationMethod=ArbitraryAxis  FollAlignAxisA=+X  BaseAlignAxisA=+Y  FollAlignAxisB=+Y  BaseAlignAxisB=+Z  RotationStandardAxis=+Z  RotationAngle=0  RotationAngleUnits=rad  RotationArbitraryAxis=[1, 0, 0]  RotationSequenceAxes=FollowerAxes  RotationSequence=XYX  RotationSequenceAngles=[0 0 0]  RotationSequenceAnglesUnits=deg  RotationMatrix=[1 0 0;0 1 0;0 0 1]  Quaternion=[1 0 0 0]  TranslationMethod=Cartesian  TranslationCartesianOffset=[0, 0, 0]  TranslationCartesianOffsetUnits=m  TranslationStandardAxis=+Z  TranslationStandardOffset=0  TranslationStandardOffsetUnits=m  TranslationROffset=0  TranslationROffsetUnits=m  TranslationThetaOffset=0  TranslationThetaOffsetUnits=deg  TranslationZOffset=0  TranslationZOffsetUnits=m
  joint3_AxisTransform : sm_lib/Frames and Transforms/Rigid Transform  RotationMethod=ArbitraryAxis  FollAlignAxisA=+X  BaseAlignAxisA=+Y  FollAlignAxisB=+Y  BaseAlignAxisB=+Z  RotationStandardAxis=+Z  RotationAngle=0  RotationAngleUnits=rad  RotationArbitraryAxis=[1, 0, 0]  RotationSequenceAxes=FollowerAxes  RotationSequence=XYX  RotationSequenceAngles=[0 0 0]  RotationSequenceAnglesUnits=deg  RotationMatrix=[1 0 0;0 1 0;0 0 1]  Quaternion=[1 0 0 0]  TranslationMethod=Cartesian  TranslationCartesianOffset=[0, 0, 0]  TranslationCartesianOffsetUnits=m  TranslationStandardAxis=+Z  TranslationStandardOffset=0  TranslationStandardOffsetUnits=m  TranslationROffset=0  TranslationROffsetUnits=m  TranslationThetaOffset=0  TranslationThetaOffsetUnits=deg  TranslationZOffset=0  TranslationZOffsetUnits=m
  joint3_OriginTransform : sm_lib/Frames and Transforms/Rigid Transform  RotationMethod=RotationSequence  FollAlignAxisA=+X  BaseAlignAxisA=+Y  FollAlignAxisB=+Y  BaseAlignAxisB=+Z  RotationStandardAxis=+Z  RotationAngle=0  RotationAngleUnits=deg  RotationArbitraryAxis=[0 0 1]  RotationSequenceAxes=BaseAxes  RotationSequence=XYZ  RotationSequenceAngles=[0, 0, 0]  RotationSequenceAnglesUnits=rad  RotationMatrix=[1 0 0;0 1 0;0 0 1]  Quaternion=[1 0 0 0]  TranslationMethod=Cartesian  TranslationCartesianOffset=[1, 0, 0]  TranslationCartesianOffsetUnits=m  TranslationStandardAxis=+Z  TranslationStandardOffset=0  TranslationStandardOffsetUnits=m  TranslationROffset=0  TranslationROffsetUnits=m  TranslationThetaOffset=0  TranslationThetaOffsetUnits=deg  TranslationZOffset=0  TranslationZOffsetUnits=m
  F : PMIOPort  Side=Left
  F1 : PMIOPort  Port=2  Side=Right
  connections:
  Inertia/RConn1 -- InertiaOriginTransform/RConn1
  ReferenceFrame/RConn1 -- InertiaOriginTransform/LConn1 -- joint2_AxisInvTransform/LConn1 -- joint3_OriginTransform/LConn1 -- VisualOriginTransform/LConn1
  Visual/RConn1 -- VisualOriginTransform/RConn1
  joint2_AxisInvTransform/RConn1 -- F/RConn1
  joint3_AxisTransform/RConn1 -- F1/RConn1
  joint3_AxisTransform/LConn1 -- joint3_OriginTransform/RConn1
